simulink model "PID_Architecture"  (R2023a)
settings: Solver=VariableStepAuto  StartTime=0.0  StopTime=200  RelTol=1e-3
undefined symbols (not defined in the file or in its folder): start_h, target_h
libraries: slpidlib x1
settings Model: Creator=HP  LastModifiedBy=HP

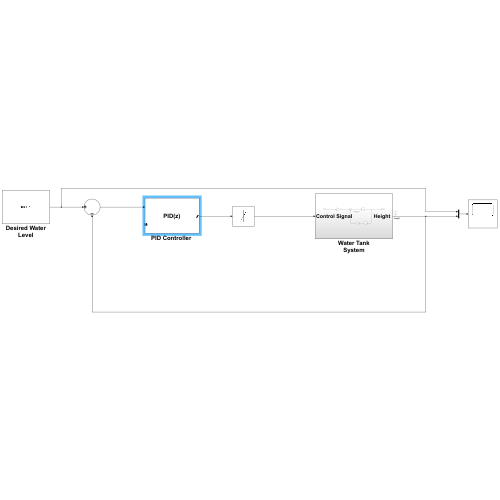
[thumbnail: Simulink's stored preview of the top-level diagram]
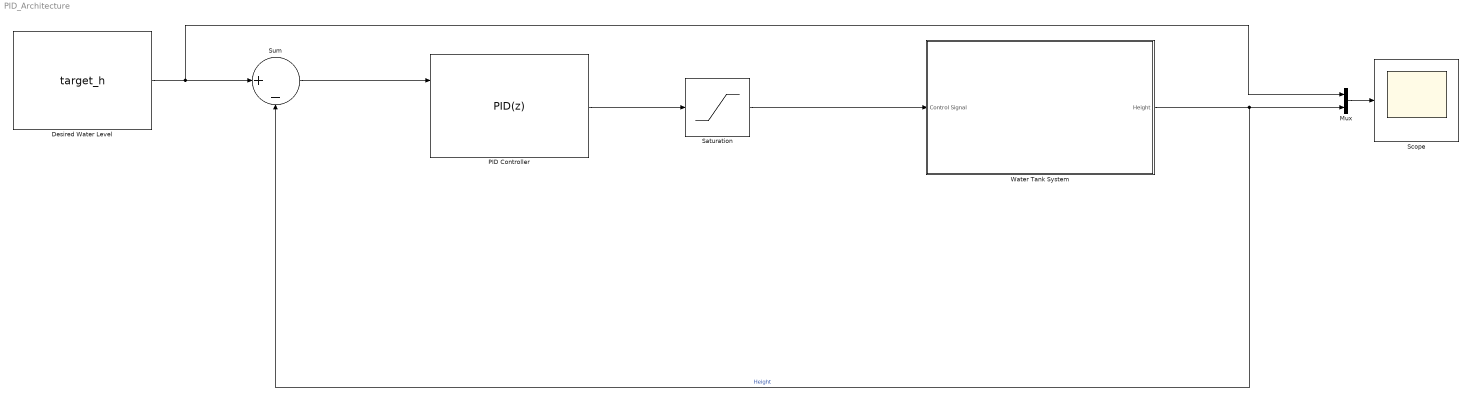
== system PID_Architecture ==
  Desired Water Level : Constant  Value=target_h
  Mux : Mux  Inputs=2
  "PID Controller " : slpidlib/PID Controller  Controller=PID  Form=Parallel  TimeDomain=Discrete-time  UseExternalTs=off  SampleTime=1  IntegratorMethod=Backward Euler  FilterMethod=Backward Euler  ControllerParametersSource=internal  P=0.778177375553426  I=0.0689945528740783  UseKiTs=off  D=-0.021110086976648  N=36.8628218545118  UseFilter=on  TunerSelectOption=Transfer Function Based (PID Tuner App)  ZeroCross=off  InitialConditionSource=internal  InitialConditionForIntegrator=0  InitialConditionForFilter=0  DifferentiatorICPrevScaledInput=0  ExternalReset=level  TrackingMode=off  Kt=1  LimitOutput=on  SatLimitsSource=internal  UpperSaturationLimit=10  LowerSaturationLimit=0  LinearizeAsGain=on  AntiWindupMode=clamping  Kb=1  LimitIntegrator=off  UpperIntegratorSaturationLimit=inf  LowerIntegratorSaturationLimit=-inf  RndMeth=Zero  POutMin=[]  POutMax=[]  IOutMin=[]  IOutMax=[]  DOutMin=[]  DOutMax=[]  NOutMin=[]  NOutMax=[]  SumOutMin=[]  SumOutMax=[]  SaturationOutMin=[]  SaturationOutMax=[]  PParamMin=[]  PParamMax=[]  IParamMin=[]  IParamMax=[]  DParamMin=[]  DParamMax=[]  NParamMin=[]  NParamMax=[]  KbParamMin=[]  KbParamMax=[]  KtParamMin=[]  KtParamMax=[]  KbOutMin=[]  KbOutMax=[]  KtOutMin=[]  KtOutMax=[]  IntegratorOutMin=[]  IntegratorOutMax=[]  FilterOutMin=[]  FilterOutMax=[]  SumI1OutMin=[]  SumI1OutMax=[]  SumI2OutMin=[]  SumI2OutMax=[]  SumI3OutMin=[]  SumI3OutMax=[]  SumI4OutMin=[]  SumI4OutMax=[]  SumDOutMin=[]  SumDOutMax=[]  DifferentiatorOutMin=[]  DifferentiatorOutMax=[]  FilterDiffOutCoefMin=[]  FilterDiffOutCoefMax=[]  ReciprocalOutMin=[]  ReciprocalOutMax=[]  SumDenOutMin=[]  SumDenOutMax=[]  SumNumOutMin=[]  SumNumOutMax=[]  DivideOutMin=[]  DivideOutMax=[]  UdiffTsProdOutMin=[]  UdiffTsProdOutMax=[]  NTsProdOutMin=[]  NTsProdOutMax=[]  UintegralTsProdOutMin=[]  UintegralTsProdOutMax=[]  UngainTsProdOutMin=[]  UngainTsProdOutMax=[]  ClampingZeroOutDataTypeStr=Inherit: Inherit via back propagation  ClampingZeroOutMin=[]  ClampingZeroOutMax=[]  FilterDenConstantOutDataTypeStr=Inherit: Inherit via back propagation  FilterDenConstantOutMin=[]  FilterDenConstantOutMax=[]  PCopyOutDataTypeStr=Inherit: Inherit via back propagation  PCopyOutMin=[]  PCopyOutMax=[]  NCopyOutDataTypeStr=Inherit: Inherit via back propagation  NCopyOutMin=[]  NCopyOutMax=[]  IntegratorContinuousStateAttributes=''  IntegratorStateMustResolveToSignalObject=off  IntegratorRTWStateStorageClass=Auto  FilterContinuousStateAttributes=''  FilterStateMustResolveToSignalObject=off  FilterRTWStateStorageClass=Auto  ParallelPVariant=InternalParameters  IdealPVariant=Disabled  IVariant=InternalParameters  DVariant=InternalParameters  IntegratorVariant=Discrete  SatVariant=Enabled  AWVariant=DiscClampingParallel  PCopyVariant=Disabled  TRVariant=Disabled  FdbkBlocksVariant=Feedback  IdealPFdbkVariant=Passthrough  SatFdbkVariant=Passthrough  DerivativeFilterVariant=BackwardEulerFilter  NVariant=InternalParameters  NCopyVariant=InternalParameters  FilterICVariant=InternalICsFilter  IntegratorICVariant=InternalICs  ExternalResetVariant=ExternalReset  TRSumVariant=Passthrough  SumFdbkVariant=Enabled  SumVariant=Sum_PID  TsampFilterVariant=InternalTs  TsampNgainVariant=Passthrough  TsampIntegralVariant=Disabled_SignalSpec  ExternalSaturationOutDataTypeStr=Inherit: Same as second input
  Saturation : Saturate  UpperLimit=10  LowerLimit=0
  Scope : Scope
  Sum : Sum  Inputs=|+-
  Water Tank System : Subsystem
  wires:
  Sum/1 -> "PID Controller "/1
  Saturation/1 -> Water Tank System/1("Control Signal ")
  "PID Controller "/1 -> Saturation/1
  Water Tank System/1("Height ") -> Sum/2, Mux/2  "Height"
  Desired Water Level/1 -> Mux/1, Sum/1
  Mux/1 -> Scope/1

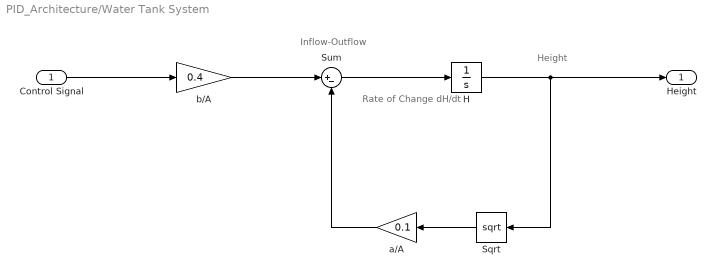
== system PID_Architecture/Water Tank System ==
  note: Inflow-Outflow
  note: Rate of Change
      | dH/dt
  note: Height
  "Control Signal " : Inport
  H : Integrator  InitialCondition=start_h  LimitOutput=on  UpperSaturationLimit=20  LowerSaturationLimit=0.001
  Sqrt : Sqrt
  Sum : Sum  Inputs=|+-
  a/A : Gain  Gain=0.1
  b/A : Gain  Gain=0.4
  "Height " : Outport
  wires:
  Sum/1 -> H/1
  "Control Signal "/1 -> b/A/1
  b/A/1 -> Sum/1
  H/1 -> "Height "/1, Sqrt/1
  a/A/1 -> Sum/2
  Sqrt/1 -> a/A/1
